simulink model "mixr_level_test"  (R2026a)
settings: Solver=FixedStepAuto  StopTime=inf  FixedStep=0.05  EnableMultiTasking=on
values from neighbouring files (symbols this model uses):
  fc_cmd = Simulink.Parameter(uint8(0)); fc_cmd.CoderInfo.StorageClass    = 'ExportedGlobal'    [init_params.m]
  fc_drainTo = Simulink.Parameter(0);  fc_drainTo.CoderInfo.StorageClass = 'ExportedGlobal'    [init_params.m]
  fc_overshoot = Simulink.Parameter(20); fc_overshoot.CoderInfo.StorageClass = 'ExportedGlobal'    [init_params.m]
  fc_pumpV = Simulink.Parameter(6);       fc_pumpV.CoderInfo.StorageClass  = 'ExportedGlobal'    [init_params.m]
  fc_settle = Simulink.Parameter(5);  fc_settle.CoderInfo.StorageClass    = 'ExportedGlobal'    [init_params.m]
  fc_target = Simulink.Parameter(50);       fc_target.CoderInfo.StorageClass = 'ExportedGlobal'    [init_params.m]
  fc_tofGain = Simulink.Parameter(1.00901);    fc_tofGain.CoderInfo.StorageClass      = 'ExportedGlobal'    [init_params.m]
  fc_tofIntercept = Simulink.Parameter(14.477);     fc_tofIntercept.CoderInfo.StorageClass = 'ExportedGlobal'    [init_params.m]
  fc_tol = Simulink.Parameter(2);  fc_tol.CoderInfo.StorageClass       = 'ExportedGlobal'    [init_params.m]
  fc_valveV = Simulink.Parameter(6); fc_valveV.CoderInfo.StorageClass  = 'ExportedGlobal'    [init_params.m]
settings Model: SimulationMode=external  ExtModeTrigDuration=2  Creator=Cyril Calo  LastModifiedBy=Cyril Calo
settings SolverCC: PositivePriorityOrder=on
settings OptimizationCC: MaxStackSize=200000
settings DebuggingCC: SubsystemReferenceDiagnosticForUnitTest=warning
settings HardwareCC: ProdBitPerLong=64.0  ProdLargestAtomicInteger=LongLong  ProdLargestAtomicFloat=Double  ProdHWDeviceType=ARM Compatible->ARM Cortex-A (64-bit)
settings RTWCC: SystemTargetFile=ert.tlc  HardwareBoard=Raspberry Pi (64bit)  TLCOptions="-aInlineSetEventsForThisBaseRateFcn=TLC_FALSE -aSuppressMultiTaskScheduler=TLC_FALSE  -aRateBasedStepFcn=0"  GenerateReport=on  Toolchain=GNU GCC RPIUtils  BuildConfiguration=Faster Runs  LaunchReport=on  Description=Embedded Coder
settings CodeAppCC: MATLABSourceComments=on
settings ERTTargetCC: ExtModeTransport=2.0  DynamicArrayContainerType=coder::array  ERTCustomFileBanners=off  SupportContinuousTime=on  SupportNonInlinedSFcns=on  SupportVariableSizeSignals=on  ModelStepFunctionPrototypeControlCompliant=off

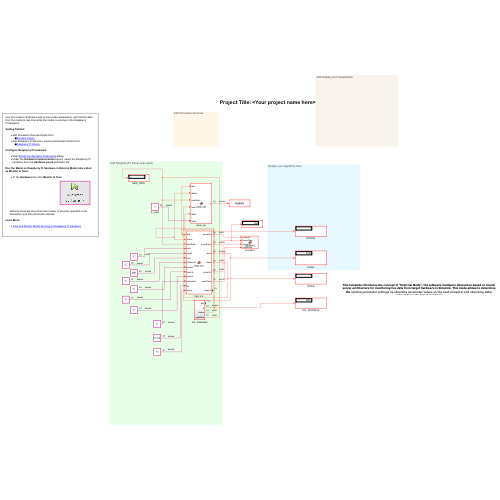
[thumbnail: Simulink's stored preview of the top-level diagram]
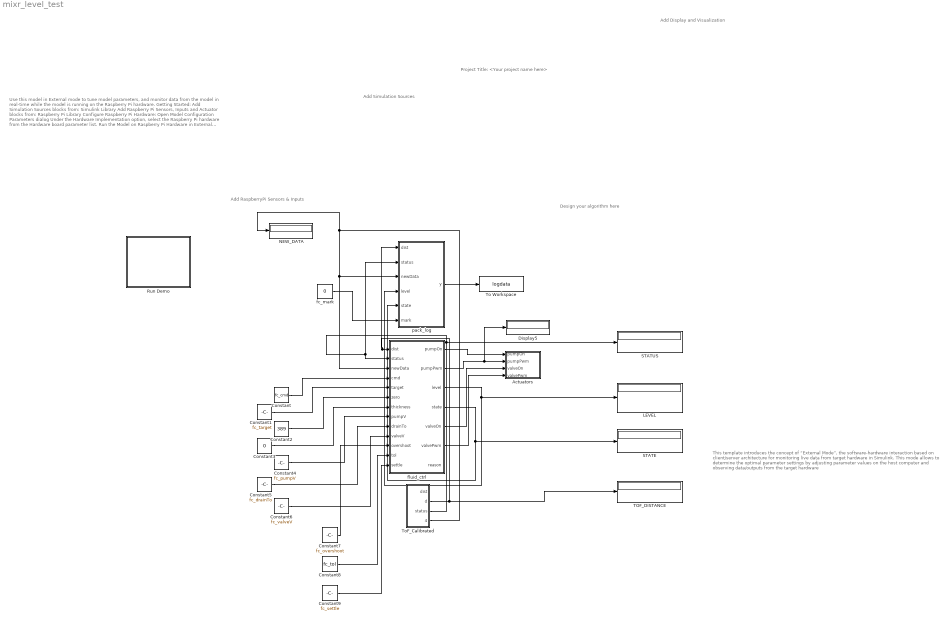
== system mixr_level_test ==
  note: Use this model in External mode to tune model parameters, and monitor data from the model in real-time while the model is running on the Raspberry Pi hardware.
      |
      | Getting Started:
      |
      | Add Simulation Sources blocks from:
      | Simulink Library
      | Add Raspberry Pi Sensors, Inputs and Actuator blocks from:
      | Raspberry Pi Library
      |
      | Configure Raspberry Pi Hardware:
      |
      | Open Model Configuration Parameters dialog
      | Under the Hardware Implementation option, select the Raspberry Pi hardware from the Hardware board parameter list.
      |
      | Run the Model on Raspberry Pi Hardware in External Mode (also called as Monitor & Tune)
      |
      | In the Hardware tab , click Monitor & Tune
      |
      | External mode will stop when the number of seconds specified in the Simulation stop time parameter elapses.
      |
      | Learn More:
      |
      | Tune and Monitor Model Running on Raspberry Pi Hardware
  note: Add Display and Visualization
  note: This template introduces the concept of “External Mode”, the software-hardware interaction based on client/server architecture for monitoring live data from target hardware in Simulink. This mode allows to determine the optimal parameter settings by adjusting parameter values on the host computer and observing data/outputs from the target hardware
  note: Design your algorithm here
  note: Add Simulation Sources
  note: Add RaspberryPi Sensors & Inputs
  note: Project Title: <Your project name here>
  Actuators : MATLAB Function  TreatAsAtomicUnit=on
  Constant : Constant  Value=fc_cmd
  Constant1 : Constant  Value=fc_target
  Constant2 : Constant  Value=389
  Constant3 : Constant  Value=0
  Constant4 : Constant  Value=fc_pumpV
  Constant5 : Constant  Value=fc_drainTo
  Constant6 : Constant  Value=fc_valveV
  Constant7 : Constant  Value=fc_overshoot
  Constant8 : Constant  Value=fc_tol
  Constant9 : Constant  Value=fc_settle
  Display5 : Display
  LEVEL : Display
  NEW_DATA : Display
  Run Demo : Subsystem  Description=Controls host-side RTDX processing.
      mask Display: pic=imread('raspberrypiMonitorAndTune.png');image(pic);
  STATE : Display
  STATUS : Display
  TOF_DISTANCE : Display
  To Workspace : ToWorkspace  VariableName=logdata  SaveFormat=Timeseries  SampleTime=-1
  ToF_Calibrated : Subsystem
  fc_mark : Constant  Value=0
  fluid_ctrl : MATLAB Function  TreatAsAtomicUnit=on
  pack_log : MATLAB Function  TreatAsAtomicUnit=on
  wires:
  Constant/1 -> fluid_ctrl/4(cmd)
  Constant1/1 -> fluid_ctrl/5(target)
  Constant2/1 -> fluid_ctrl/6(zero)
  Constant3/1 -> fluid_ctrl/7(thickness)
  Constant4/1 -> fluid_ctrl/8(pumpV)
  fluid_ctrl/3(level) -> pack_log/4(level), LEVEL/1
  fluid_ctrl/4(state) -> pack_log/5(state), STATE/1
  fluid_ctrl/1(pumpOn) -> Actuators/1(pumpOn)
  fluid_ctrl/2(pumpPwm) -> Display5/1, Actuators/2(pumpPwm)
  fc_mark/1 -> pack_log/6(mark)
  pack_log/1(y) -> To Workspace/1
  Constant5/1 -> fluid_ctrl/9(drainTo)
  Constant6/1 -> fluid_ctrl/10(valveV)
  fluid_ctrl/5(valveOn) -> Actuators/3(valveOn)
  fluid_ctrl/6(valvePwm) -> Actuators/4(valvePwm)
  Constant7/1 -> fluid_ctrl/11(overshoot)
  Constant8/1 -> fluid_ctrl/12(tol)
  Constant9/1 -> fluid_ctrl/13(settle)
  ToF_Calibrated/4(newData) -> fluid_ctrl/3(newData), pack_log/3(newData), NEW_DATA/1
  ToF_Calibrated/3(status) -> pack_log/2(status), fluid_ctrl/2(status), STATUS/1
  ToF_Calibrated/2(d) -> TOF_DISTANCE/1, pack_log/1(dist), fluid_ctrl/1(dist)

== system mixr_level_test/Run Demo ==

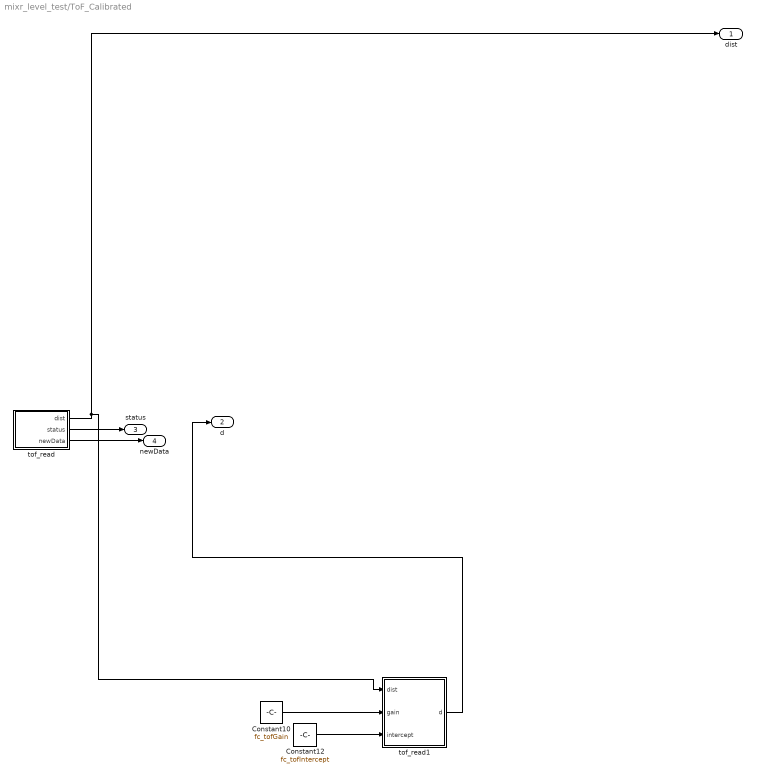
== system mixr_level_test/ToF_Calibrated ==
  Constant10 : Constant  Value=fc_tofGain
  Constant12 : Constant  Value=fc_tofIntercept
  tof_read : MATLAB Function  TreatAsAtomicUnit=on
  tof_read1 : MATLAB Function  TreatAsAtomicUnit=on
  dist : Outport
  d : Outport  Port=2
  status : Outport  Port=3
  newData : Outport  Port=4
  wires:
  tof_read1/1(d) -> d/1
  tof_read/1(dist) -> dist/1, tof_read1/1(dist)
  Constant12/1 -> tof_read1/3(intercept)
  Constant10/1 -> tof_read1/2(gain)
  tof_read/2(status) -> status/1
  tof_read/3(newData) -> newData/1

== matlab function mixr_level_test/Actuators ==
  data: pumpOn input; pumpPwm input; valveOn input; valvePwm input
function actuators(pumpOn, pumpPwm, valveOn, valvePwm) %#codegen
coder.extrinsic('which', 'fileparts');
persistent started
if isempty(started), started = false; end
if ~coder.target('Sfun')
    srcDir = coder.const(fileparts(which('act_wrapper.c')));
    coder.cinclude('act_wrapper.h');
    coder.updateBuildInfo('addIncludePaths', srcDir);
    coder.updateBuildInfo('addSourcePaths',  srcDir);
    coder.updateBuildInfo('addSourceFiles', 'act_wrapper.c');
    coder.updateBuildInfo('addLinkFlags', '-lwiringPi');
    if ~started
        coder.ceval('act_init');
        started = true;
    end
    coder.ceval('act_step', pumpOn, pumpPwm, valveOn, valvePwm);
end
end

== matlab function mixr_level_test/ToF_Calibrated/tof_read ==
  data: dist output; status output; newData output
function [dist, status, newData] = tof_read() %#codegen
coder.extrinsic('which', 'fileparts');
dist    = uint16(0);
status  = uint8(255);
newData = uint8(0);

persistent k started
if isempty(k)
    k = uint16(0);
    started = false;
end

if coder.target('Sfun')
    dist    = uint16(150) - mod(k, uint16(100));
    k       = k + uint16(1);
    status  = uint8(0);
    newData = uint8(1);
else
    srcDir = coder.const(fileparts(which('tof_wrapper.c')));
    coder.cinclude('tof_wrapper.h');
    coder.updateBuildInfo('addIncludePaths', srcDir);
    coder.updateBuildInfo('addSourcePaths',  srcDir);
    coder.updateBuildInfo('addSourceFiles', 'tof_wrapper.c');
    coder.updateBuildInfo('addSourceFiles', 'VL53L4CD_api.c');
    coder.updateBuildInfo('addSourceFiles', 'platform.c');

    if ~started
        coder.ceval('tof_init', int16(-26), uint16(200));
        started = true;
    end
    coder.ceval('tof_step', coder.wref(dist), coder.wref(status), coder.wref(newData));
end
end

== matlab function mixr_level_test/fluid_ctrl ==
  data: pumpOn output; pumpPwm output; level output; dist input; status input; newData input; cmd input; target input; zero input; thickness input; pumpV input; state output; drainTo input; valveV input; valveOn output; valvePwm output; overshoot input; tol input; settle input; reason output
function [pumpOn, pumpPwm, level, state, valveOn, valvePwm, reason] = fluid_ctrl( ...
        dist, status, newData, cmd, target, zero, thickness, pumpV, drainTo, valveV, ...
        overshoot, tol, settle) %#codegen
% cmd:   0 idle, 1 fill, 2 drain, 3 feedback fill, 4 go to target by settling,
%        5 manual drain, 6 manual pump, 7 hysteresis (valve always open, pump between low and target)
%        Any new command goes to state 0 first, then starts.
% state: 0 idle, 1 filling, 2 draining, 3 in band (keeps regulating while hold = 1),
%        4 drain done, 5 overfill, 6 settling, 7 trim-drain, 8 trim-fill, 9 fault,
%        11 manual drain, 12 manual pump, 13 hysteresis drain-down, 14 hysteresis refill
% reason (when state is 9): 1 no sensor frames, 2 invalid readings, 3 phase timeout
% live values: react, hold, low (hysteresis pump-on level, 0 = target - 10)
coder.extrinsic('which', 'fileparts');
DT         = 0.05;    % model step size in seconds (Solver: fixed-step 0.05)
GAP_STEPS  = 2;       % steps in state 0 between a new command and its start
N_MED      = 3;       % level filter length: 1 = fastest response, 3 = smoother
MAX_AGE    = 12;      % outputs stay off if the last sensor frame is older than 12 steps
EMPTY_MM   = 2.0;     % automatic drain never goes below this
MAX_BAD    = 10;      % consecutive invalid frames while pumping/draining -> fault
MAX_SILENT = 40;      % steps with no new frame while pumping/draining -> fault (2 s)
MAX_RUN    = 4800;    % max steps for one pump or valve phase (240 s)
BIG_MM     = 10;      % errors larger than this are corrected at full power
BACKOFF    = 0.7;     % each failed correction in a row uses 70% of the previous power
SCALE_MIN  = 0.2;     % never go below 20% of the commanded power
V_MAX      = 24.0;    % supply voltage: pumpV and valveV are the average volts at the load
PWM_RANGE  = 1024;

persistent st prevSt prevCmd prevSeq buf nvalid bad silent runSteps outSteps fails curScale ...
           lvl haveLvl why pending gap ctlStarted
if isempty(st)
    st = uint8(0); prevSt = uint8(0); prevCmd = uint8(0); prevSeq = 0;
    buf = zeros(1,3); nvalid = 0; bad = 0; silent = 0; runSteps = 0; outSteps = 0;
    fails = 0; curScale = 1; lvl = 0; haveLvl = false;
    why = uint8(0); pending = uint8(0); gap = 0; ctlStarted = false;
end

% ---- live control values (UDP overrides the Constant blocks) ----
defs = [double(cmd), target, pumpV, valveV, drainTo, overshoot, tol, settle, zero, thickness, ...
        1.0, 0.0, 1.0, 1.0, 1.0, 0.0, 0.0];
vals = defs;
if ~coder.target('Sfun')
    srcDir = coder.const(fileparts(which('ctl_wrapper.c')));
    coder.cinclude('ctl_wrapper.h');
    coder.updateBuildInfo('addIncludePaths', srcDir);
    coder.updateBuildInfo('addSourcePaths',  srcDir);
    coder.updateBuildInfo('addSourceFiles', 'ctl_wrapper.c');
    if ~ctlStarted
        coder.ceval('ctl_init');
        ctlStarted = true;
    end
    coder.ceval('ctl_poll', coder.rref(defs), coder.wref(vals));
end
c   = uint8(min(max(round(vals(1)), 0), 255));
tgt = vals(2);  pV = vals(3);  vV = vals(4);  dTo = vals(5);
ovs = vals(6);  tl = vals(7);  stl = vals(8);  z0 = vals(9);  th = vals(10);
lg  = vals(11);                     % level scale
ld  = max(vals(12), 0);             % lead: stop this many mm early to cancel coasting
ts  = min(max(vals(13), 0), 1);     % trim power scale
rc  = max(vals(14), 0.2);           % react: seconds out of band before state 3 corrects
hd  = vals(15) >= 0.5;              % hold: 1 = state 3 keeps regulating
lowRaw = vals(16);                  % hysteresis: pump switches on at or below this level
sq  = vals(17);                     % number of command messages received
settleSteps = round(stl / DT);
reactSteps  = round(rc / DT);
if lowRaw <= 0
    lowEff = tgt - 10;
else
    lowEff = lowRaw;
end
lowEff = min(lowEff, tgt - max(tl, 2));     % keep a gap of at least the tolerance

% ---- new sensor frame ----
if newData == 1
    silent = 0;
    if status == 0 && dist > 30 && dist <= 2000
        buf = [buf(2:3), double(dist)];
        nvalid = min(nvalid + 1, 3);
        bad = 0;
        nuse = min(nvalid, N_MED);
        lvl = max(0, lg * (z0 - median(buf(4-nuse:3)) - th));
        haveLvl = true;
    else
        bad = bad + 1;
    end
else
    silent = min(silent + 1, 1e6);
end

% ---- commands: any new command goes to state 0 first, then starts ----
newCmd = (c ~= prevCmd) || (sq ~= prevSeq);
if c == 0
    st = uint8(0);
    why = uint8(0); pending = uint8(0); gap = 0;
elseif newCmd && c <= 7
    st = uint8(0);                              % everything off (also clears a fault)
    why = uint8(0);
    pending = c; gap = GAP_STEPS;
    bad = 0; runSteps = 0; outSteps = 0; fails = 0; curScale = 1;
elseif pending ~= 0
    gap = gap - 1;
    if gap <= 0
        if pending == 3
            st = uint8(5);
        elseif pending == 4
            st = uint8(6);
        elseif pending == 5
            st = uint8(11);
        elseif pending == 6
            st = uint8(12);
        elseif pending == 7
            st = uint8(13);
        else
            st = pending;                       % 1 fill, 2 drain
        end
        pending = uint8(0);
    end
end
prevCmd = c;
prevSeq = sq;

% ---- count steps spent in the current phase ----
if st ~= prevSt
    runSteps = 0;
end
prevSt = st;
ok = haveLvl && silent <= MAX_AGE;

% ---- automatic modes ----
pumping  = (st == 1 || st == 5 || st == 8 || st == 14);
draining = (st == 2 || st == 7 || st == 13 || st == 14);
if pumping || draining
    runSteps = runSteps + 1;
    limit = MAX_RUN;
    if st == 13, limit = 4 * MAX_RUN; end       % a slow drain-down may take longer
    if bad >= MAX_BAD
        st = uint8(9); why = uint8(2);
    elseif silent >= MAX_SILENT
        st = uint8(9); why = uint8(1);
    elseif runSteps >= limit
        st = uint8(9); why = uint8(3);
    elseif haveLvl
        if st == 1
            if lvl >= tgt - ld, st = uint8(3); outSteps = 0; end
        elseif st == 2
            if lvl <= max(dTo, EMPTY_MM), st = uint8(4); end
        elseif st == 5
            if lvl >= tgt + max(ovs, 0) - ld, st = uint8(6); end
        elseif st == 7
            if lvl <= tgt + ld, st = uint8(6); end
        elseif st == 8
            if lvl >= tgt - ld, st = uint8(6); end
        elseif st == 13
            if lvl <= lowEff, st = uint8(14); end       % low level reached: pump on
        elseif st == 14
            if lvl >= tgt - ld, st = uint8(13); end     % target reached: pump off, drain continues
        end
    end
elseif st == 6
    runSteps = runSteps + 1;
    if ok && runSteps >= settleSteps
        err = lvl - tgt;
        if abs(err) <= tl
            st = uint8(3); fails = 0; outSteps = 0;
        else
            fails = fails + 1;
            if abs(err) > BIG_MM
                curScale = 1;
            else
                curScale = max(SCALE_MIN, ts * BACKOFF^(fails - 1));
            end
            if err > 0
                st = uint8(7);
            else
                st = uint8(8);
            end
        end
    end
elseif st == 3 && hd
    % continuous regulation: react when the level has been outside the band for react seconds
    if ok && abs(lvl - tgt) > tl
        outSteps = outSteps + 1;
    else
        outSteps = max(0, outSteps - 2);        % in-band readings drain the counter, not reset it
    end
    if outSteps >= reactSteps
        outSteps = 0; fails = 1;
        err = lvl - tgt;
        if abs(err) > BIG_MM
            curScale = 1;
        else
            curScale = max(SCALE_MIN, ts);
        end
        if err > 0
            st = uint8(7);
        else
            st = uint8(8);
        end
    end
end

% ---- manual modes (run without a level reading) ----
if st == 11 || st == 12
    runSteps = runSteps + 1;
    if runSteps >= MAX_RUN
        st = uint8(9); why = uint8(3);
    elseif st == 12 && haveLvl && lvl >= tgt + max(ovs, 0)
        st = uint8(4);              % ceiling reached, pump stops
    end
end

% ---- outputs ----
ok      = haveLvl && silent <= MAX_AGE;
pumpOn  = uint8(((st == 1 || st == 5 || st == 8 || st == 14) && ok) || st == 12);
valveOn = uint8(((st == 2 || st == 7 || st == 13 || st == 14) && ok) || st == 11);
scale = 1.0;
if st == 7 || st == 8, scale = curScale; end
pumpPwm  = uint16(min(PWM_RANGE, max(0, round(scale * pV / V_MAX * PWM_RANGE))));
valvePwm = uint16(min(PWM_RANGE, max(0, round(scale * vV / V_MAX * PWM_RANGE))));
level    = lvl;
state    = st;
reason   = why;
end

== matlab function mixr_level_test/pack_log ==
  data: y output; dist input; status input; newData input; level input; state input; mark input
function y = pack_log(dist, status, newData, level, state, mark) %#codegen
y = [double(dist), double(status), double(newData), level, double(state), mark];
end

== matlab function mixr_level_test/ToF_Calibrated/tof_read1 ==
  data: d output; dist input; gain input; intercept input
function d = tof_correct(dist, gain, intercept) %#codegen
% same formula as tofCorrect() in tof_cal.cpp: corrected = (raw - b) / m
if dist == 0
    d = 0;                        % no reading yet, pass through
else
    d = (double(dist) - intercept) / gain;
end
end
